simulink model "ASM_Traffic_new"  (R2024a)
settings: Solver=ode1  StartTime=SIM.tstart.v  StopTime=SIM.tend.v  FixedStep=SIM.StepSize.v  RelTol=1e-3
PostLoadFcn:
  | if any(exist('dsrtsu_mdlpostloadfcn', 'file') ~= 0), dsrtsu_mdlpostloadfcn('Execute', bdroot); end
  | try, asm_mdl_postloadfcn(bdroot, 'UpdateModel', 3600); catch, disp(lasterr); end,
InitFcn:
  | , if any(exist('rtifpga_mdlclblib', 'file') ~= 0), rtifpga_mdlclblib('Init', bdroot); end,
  | , if any(exist('dsmpb_private', 'file') ~= 0), dsmpb_private('dsmpb_mdlclblib', 'Init', bdroot); end,
undefined symbols (not defined in the file): _to_, a0b2, ASM_BrakeHydraulics_DemoSystems, ASM_VehicleDynamics_DemoSystems, b98103fe8ad365046cd0, BrakeCircuit, CPT, Crankshaft, DiscIntNeverNeededParam, dsmsi, FinalDriveAssembly, MDL, ModeSignals, Pos_BrakePedal_Maneuver, rad, RefSignals, s_to_rpm, SIM, SoftECU, Suspension, Tire, Transmission
libraries: ASM_Traffic_lib x135, simulink x100, ASM_Utils_lib x77, ASM_VehicleDynamics_lib x70, ASM_Environment_lib x22, dsmpblib x20, dsmsilib x15, MDLD_Utils_lib x10, ASM_BrakeHydraulics_lib x3
(part 42 of 63)

== system ASM_Traffic_new/VehicleDynamics/Plant/UserInterface/DISP_Plant/Aerodynamics ==
  Aerodynamics : Inport
  Aerodynamics1 : Scope  NumInputPorts=2
  Bus Selector5 : BusSelector  OutputSignals=Forces.F_x_Aero_CoorSys_V[N],Forces.F_y_Aero_CoorSys_V[N],Forces.F_z_Aero_CoorSys_V[N],Torques.Trq_x_Aero_CoorSys_V[Nm],Torques.Trq_y_Aero_CoorSys_V[Nm],Torques.Trq_z_Aero_CoorSys_V[Nm]
  F_x_Aero_CoorSys_V[N] : Subsystem
      mask Display: disp('')
  F_y_Aero_CoorSys_V[N] : Subsystem
      mask Display: disp('')
  F_z_Aero_CoorSys_V[N] : Subsystem
      mask Display: disp('')
  Mux : Mux  Inputs=3
  Mux1 : Mux  Inputs=3
  Trq_x_Aero_CoorSys_V[Nm] : Subsystem
      mask Display: disp('')
  Trq_y_Aero_CoorSys_V[Nm] : Subsystem
      mask Display: disp('')
  Trq_z_Aero_CoorSys_V[Nm] : Subsystem
      mask Display: disp('')
  wires:
  Trq_z_Aero_CoorSys_V[Nm]/1(Out1) -> Mux1/3  "Trq_z_Aero_CoorSys_V[Nm]"
  Bus Selector5/6 -> Trq_z_Aero_CoorSys_V[Nm]/1(In1)  "<Trq_z_Aero_CoorSys_V[Nm]>"
  Trq_y_Aero_CoorSys_V[Nm]/1(Out1) -> Mux1/2  "Trq_y_Aero_CoorSys_V[Nm]"
  Bus Selector5/5 -> Trq_y_Aero_CoorSys_V[Nm]/1(In1)  "<Trq_y_Aero_CoorSys_V[Nm]>"
  Trq_x_Aero_CoorSys_V[Nm]/1(Out1) -> Mux1/1  "Trq_x_Aero_CoorSys_V[Nm]"
  Bus Selector5/4 -> Trq_x_Aero_CoorSys_V[Nm]/1(In1)  "<Trq_x_Aero_CoorSys_V[Nm]>"
  F_z_Aero_CoorSys_V[N]/1(Out1) -> Mux/3  "F_z_Aero_CoorSys_V[N]"
  Bus Selector5/3 -> F_z_Aero_CoorSys_V[N]/1(In1)  "<F_z_Aero_CoorSys_V[N]>"
  F_y_Aero_CoorSys_V[N]/1(Out1) -> Mux/2  "F_y_Aero_CoorSys_V[N]"
  Bus Selector5/2 -> F_y_Aero_CoorSys_V[N]/1(In1)  "<F_y_Aero_CoorSys_V[N]>"
  F_x_Aero_CoorSys_V[N]/1(Out1) -> Mux/1  "F_x_Aero_CoorSys_V[N]"
  Bus Selector5/1 -> F_x_Aero_CoorSys_V[N]/1(In1)  "<F_x_Aero_CoorSys_V[N]>"
  Mux1/1 -> Aerodynamics1/2  "Trq_Aero[Nm]"
  Mux/1 -> Aerodynamics1/1  "F_Aero[N]"
  Aerodynamics/1 -> Bus Selector5/1

== system ASM_Traffic_new/VehicleDynamics/Plant/UserInterface/DISP_Plant/Brake ==
  Brake : Inport
  BrakeHydraulicsModel : Display
      settings: AttributesFormatString=1 - Complex\n2 - Basic
  BrakeHydraulicsModel[] : Subsystem
      mask Display: disp('')
  BrakePressure : Scope  NumInputPorts=6
  BrakeTorques : Scope  NumInputPorts=4
  Bus Selector2 : BusSelector  OutputSignals=BrakeHydraulics.BrakeHydraulicsModel[],BrakeDisc.Torque.Trq_FL_Brake[Nm],BrakeDisc.Torque.Trq_FR_Brake[Nm],BrakeDisc.Torque.Trq_RL_Brake[Nm],BrakeDisc.Torque.Trq_RR_Brake[Nm],MasterBrakeCylinder.ActiveBrakeCylinder.p[bar],MasterBrakeCylinder.ActiveBrakeCylinder.p_max[bar],BrakeDisc.Pressure.p_FL_Brake[bar],BrakeDisc.Pressure.p_FR_Brake[bar],BrakeDisc.Pressure.p_RL_Brake[bar],BrakeDisc.Pressure.p_RR_Brake[bar]
  Trq_FL_Brake[Nm] : Subsystem
      mask Display: disp('')
  Trq_FR_Brake[Nm] : Subsystem
      mask Display: disp('')
  Trq_RL_Brake[Nm] : Subsystem
      mask Display: disp('')
  Trq_RR_Brake[Nm] : Subsystem
      mask Display: disp('')
  p[bar] : Subsystem
      mask Display: disp('')
  p_FL_Brake[bar] : Subsystem
      mask Display: disp('')
  p_FR_Brake[bar] : Subsystem
      mask Display: disp('')
  p_RL_Brake[bar] : Subsystem
      mask Display: disp('')
  p_RR_Brake[bar] : Subsystem
      mask Display: disp('')
  p_max[bar] : Subsystem
      mask Display: disp('')
  wires:
  p_RR_Brake[bar]/1(Out1) -> BrakePressure/6  "p_RR_Brake[bar]"
  Bus Selector2/11 -> p_RR_Brake[bar]/1(In1)  "<p_RR_Brake[bar]>"
  p_RL_Brake[bar]/1(Out1) -> BrakePressure/5  "p_RL_Brake[bar]"
  Bus Selector2/10 -> p_RL_Brake[bar]/1(In1)  "<p_RL_Brake[bar]>"
  p_FR_Brake[bar]/1(Out1) -> BrakePressure/4  "p_FR_Brake[bar]"
  Bus Selector2/9 -> p_FR_Brake[bar]/1(In1)  "<p_FR_Brake[bar]>"
  p_FL_Brake[bar]/1(Out1) -> BrakePressure/3  "p_FL_Brake[bar]"
  Bus Selector2/8 -> p_FL_Brake[bar]/1(In1)  "<p_FL_Brake[bar]>"
  p_max[bar]/1(Out1) -> BrakePressure/2  "p_max[bar]"
  Bus Selector2/7 -> p_max[bar]/1(In1)  "<p_max[bar]>"
  p[bar]/1(Out1) -> BrakePressure/1  "p[bar]"
  Bus Selector2/6 -> p[bar]/1(In1)  "<p[bar]>"
  Trq_RR_Brake[Nm]/1(Out1) -> BrakeTorques/4  "Trq_RR_Brake[Nm]"
  Bus Selector2/5 -> Trq_RR_Brake[Nm]/1(In1)  "<Trq_RR_Brake[Nm]>"
  Trq_RL_Brake[Nm]/1(Out1) -> BrakeTorques/3  "Trq_RL_Brake[Nm]"
  Bus Selector2/4 -> Trq_RL_Brake[Nm]/1(In1)  "<Trq_RL_Brake[Nm]>"
  Trq_FR_Brake[Nm]/1(Out1) -> BrakeTorques/2  "Trq_FR_Brake[Nm]"
  Bus Selector2/3 -> Trq_FR_Brake[Nm]/1(In1)  "<Trq_FR_Brake[Nm]>"
  Trq_FL_Brake[Nm]/1(Out1) -> BrakeTorques/1  "Trq_FL_Brake[Nm]"
  Bus Selector2/2 -> Trq_FL_Brake[Nm]/1(In1)  "<Trq_FL_Brake[Nm]>"
  Brake/1 -> Bus Selector2/1
  BrakeHydraulicsModel[]/1(Out1) -> BrakeHydraulicsModel/1  "BrakeHydraulicsModel[]"
  Bus Selector2/1 -> BrakeHydraulicsModel[]/1(In1)  "<BrakeHydraulicsModel[]>"

== system ASM_Traffic_new/VehicleDynamics/Plant/UserInterface/DISP_Plant/Overview ==
  Velocities : Inport
  Accelerations : Inport  Port=2
  Bus Selector1 : BusSelector  OutputSignals=VehicleCoG.Linear.a_Vehicle_CoG[x;y;z][m|s2].a_x_Vehicle_CoG[m|s2],VehicleCoG.Linear.a_Vehicle_CoG[x;y;z][m|s2].a_y_Vehicle_CoG[m|s2],VehicleCoG.Linear.a_Vehicle_CoG[x;y;z][m|s2].a_z_Vehicle_CoG[m|s2]
  Bus Selector2 : BusSelector  OutputSignals=Vehicle.Linear.v_Vehicle_CoG[x;y;z][km|h].v_x_Vehicle_CoG[km|h],Vehicle.Linear.v_Vehicle_CoG[x;y;z][km|h].v_y_Vehicle_CoG[km|h],Vehicle.Linear.v_Vehicle_CoG[x;y;z][km|h].v_z_Vehicle_CoG[km|h],Vehicle.Linear.v_Total_Vehicle[km|h]
  Mux : Mux
  Mux1 : Mux  Inputs=3
  Overview : Scope  NumInputPorts=2
  a_x_Vehicle_CoG[m|s2] : Subsystem
      mask Display: disp('')
  a_y_Vehicle_CoG[m|s2] : Subsystem
      mask Display: disp('')
  a_z_Vehicle_CoG[m|s2] : Subsystem
      mask Display: disp('')
  v_Total_Vehicle[km|h] : Subsystem
      mask Display: disp('')
  v_x_Vehicle_CoG[km|h] : Subsystem
      mask Display: disp('')
  v_y_Vehicle_CoG[km|h] : Subsystem
      mask Display: disp('')
  v_z_Vehicle_CoG[km|h] : Subsystem
      mask Display: disp('')
  wires:
  Velocities/1 -> Bus Selector2/1
  Accelerations/1 -> Bus Selector1/1
  Mux/1 -> Overview/1  "Velocities"
  Mux1/1 -> Overview/2  "Accelerations"
  v_x_Vehicle_CoG[km|h]/1(Out1) -> Mux/1  "v_x_Vehicle_CoG[km|h]"
  v_y_Vehicle_CoG[km|h]/1(Out1) -> Mux/2  "v_y_Vehicle_CoG[km|h]"
  v_z_Vehicle_CoG[km|h]/1(Out1) -> Mux/3  "v_z_Vehicle_CoG[km|h]"
  v_Total_Vehicle[km|h]/1(Out1) -> Mux/4  "v_Total_Vehicle[km|h]"
  a_x_Vehicle_CoG[m|s2]/1(Out1) -> Mux1/1  "a_x_Vehicle_CoG[m|s2]"
  a_y_Vehicle_CoG[m|s2]/1(Out1) -> Mux1/2  "a_y_Vehicle_CoG[m|s2]"
  a_z_Vehicle_CoG[m|s2]/1(Out1) -> Mux1/3  "a_z_Vehicle_CoG[m|s2]"
  Bus Selector2/1 -> v_x_Vehicle_CoG[km|h]/1(In1)  "<v_x_Vehicle_CoG[km|h]>"
  Bus Selector2/2 -> v_y_Vehicle_CoG[km|h]/1(In1)  "<v_y_Vehicle_CoG[km|h]>"
  Bus Selector2/3 -> v_z_Vehicle_CoG[km|h]/1(In1)  "<v_z_Vehicle_CoG[km|h]>"
  Bus Selector2/4 -> v_Total_Vehicle[km|h]/1(In1)  "<v_Total_Vehicle[km|h]>"
  Bus Selector1/1 -> a_x_Vehicle_CoG[m|s2]/1(In1)  "<a_x_Vehicle_CoG[m|s2]>"
  Bus Selector1/2 -> a_y_Vehicle_CoG[m|s2]/1(In1)  "<a_y_Vehicle_CoG[m|s2]>"
  Bus Selector1/3 -> a_z_Vehicle_CoG[m|s2]/1(In1)  "<a_z_Vehicle_CoG[m|s2]>"

== system ASM_Traffic_new/VehicleDynamics/Plant/UserInterface/DISP_Plant/Positions ==
  Positions : Inport
  Angle_Pitch_Vehicle_CoorSys_E[deg] : Subsystem
      mask Display: disp('')
  Angle_Roll_Vehicle_CoorSys_E[deg] : Subsystem
      mask Display: disp('')
  Angle_Yaw_Vehicle_CoorSys_E[deg] : Subsystem
      mask Display: disp('')
  AngularPosition : Scope  NumInputPorts=3
  Bus Selector2 : BusSelector  OutputSignals=Vehicle.Linear.Pos_Vehicle_CoorSys_E[m],Vehicle.Linear.s_Vehicle[m],Vehicle.Angular.Angle_V[Alpha;Beta;Gamma][deg]
  Demux : Demux  Outputs=3
  Demux1 : Demux  Outputs=3
  Pos_x_Vehicle_CoorSys_E[m] : Subsystem
      mask Display: disp('')
  Pos_y_Vehicle_CoorSys_E[m] : Subsystem
      mask Display: disp('')
  Pos_z_Vehicle_CoorSys_E[m] : Subsystem
      mask Display: disp('')
  TransPosition : Scope  NumInputPorts=4
  s_Vehicle[m] : Subsystem
      mask Display: disp('')
  wires:
  Positions/1 -> Bus Selector2/1
  Angle_Roll_Vehicle_CoorSys_E[deg]/1(Out1) -> AngularPosition/1  "Angle_Roll_Vehicle_CoorSys_E[deg]"
  Angle_Pitch_Vehicle_CoorSys_E[deg]/1(Out1) -> AngularPosition/2  "Angle_Pitch_Vehicle_CoorSys_E[deg]"
  Angle_Yaw_Vehicle_CoorSys_E[deg]/1(Out1) -> AngularPosition/3  "Angle_Yaw_Vehicle_CoorSys_E[deg]"
  Pos_x_Vehicle_CoorSys_E[m]/1(Out1) -> TransPosition/1  "Pos_x_Vehicle_CoorSys_E[m]"
  Pos_y_Vehicle_CoorSys_E[m]/1(Out1) -> TransPosition/2  "Pos_y_Vehicle_CoorSys_E[m]"
  Pos_z_Vehicle_CoorSys_E[m]/1(Out1) -> TransPosition/3  "Pos_z_Vehicle_CoorSys_E[m]"
  s_Vehicle[m]/1(Out1) -> TransPosition/4  "s_Vehicle[m]"
  Bus Selector2/1 -> Demux/1  "<Pos_Vehicle_CoorSys_E[m]>"
  Bus Selector2/2 -> s_Vehicle[m]/1(In1)  "<s_Vehicle[m]>"
  Demux/1 -> Pos_x_Vehicle_CoorSys_E[m]/1(In1)
  Demux/2 -> Pos_y_Vehicle_CoorSys_E[m]/1(In1)
  Demux/3 -> Pos_z_Vehicle_CoorSys_E[m]/1(In1)
  Demux1/2 -> Angle_Pitch_Vehicle_CoorSys_E[deg]/1(In1)
  Demux1/1 -> Angle_Roll_Vehicle_CoorSys_E[deg]/1(In1)
  Demux1/3 -> Angle_Yaw_Vehicle_CoorSys_E[deg]/1(In1)
  Bus Selector2/3 -> Demux1/1  "<Angle_V[Alpha;Beta;Gamma][deg]>"

== system ASM_Traffic_new/VehicleDynamics/Plant/UserInterface/DISP_Plant/Sensor1 ==
  Sensor1 : Inport
  AngularAccelerations : Scope
  AngularVelocity : Scope
  AngularVelocity_CoorSys_VH : Scope
  Bus Selector2 : BusSelector  OutputSignals=a_Angular_Sensor1_CoorSys_V[x;y;z][rad|s2],a_Total_Sensor1_CoorSys_V[x;y;z][m|s2],a_Sensor1_CoorSys_V[x;y;z][m|s2],v_Sensor1_CoorSys_V[x;y;z][m|s],w_Sensor1_CoorSys_V[x;y;z][rad|s],a_Angular_Sensor1_CoorSys_VH[x;y;z][rad|s2],a_Total_Sensor1_CoorSys_VH[x;y;z][m|s2],a_Sensor1_CoorSys_VH[x;y;z][m|s2],v_Sensor1_CoorSys_VH[x;y;z][m|s],w_Sensor1_CoorSys_VH[x;y;z][rad|s]
  TransAccelerations_CoorSys_VH : Scope
  TransAccelerations_withGravity : Scope
  TransAccelerations_withGravity_CoorSys_VH : Scope
  TransAccelerations_withoutGravity : Scope
  TransAccelerations_withoutGravity_CoorSys_VH : Scope
  TransVelocity : Scope
  TransVelocity_CoorSys_VH : Scope
  a_Angular_Sensor1_CoorSys_VH[x;y;z][rad|s2] : Subsystem
      mask Display: disp('')
  a_Angular_Sensor1_CoorSys_V[x;y;z][rad|s2] : Subsystem
      mask Display: disp('')
  a_Sensor1_CoorSys_VH[x;y;z][m|s2] : Subsystem
      mask Display: disp('')
  a_Sensor1_CoorSys_V[x;y;z][m|s2] : Subsystem
      mask Display: disp('')
  a_Total_Sensor1_CoorSys_VH[x;y;z][m|s2] : Subsystem
      mask Display: disp('')
  a_Total_Sensor1_CoorSys_V[x;y;z][m|s2] : Subsystem
      mask Display: disp('')
  v_Sensor1_CoorSys_VH[x;y;z][m|s] : Subsystem
      mask Display: disp('')
  v_Sensor1_CoorSys_V[x;y;z][m|s] : Subsystem
      mask Display: disp('')
  w_Sensor1_CoorSys_VH[x;y;z][rad|s] : Subsystem
      mask Display: disp('')
  w_Sensor1_CoorSys_V[x;y;z][rad|s] : Subsystem
      mask Display: disp('')
  wires:
  Bus Selector2/9 -> v_Sensor1_CoorSys_VH[x;y;z][m|s]/1(In1)  "<v_Sensor1_CoorSys_VH[x;y;z][m|s]>"
  v_Sensor1_CoorSys_VH[x;y;z][m|s]/1(Out1) -> TransVelocity_CoorSys_VH/1  "v_Sensor1_CoorSys_VH[x;y;z][m|s]"
  w_Sensor1_CoorSys_VH[x;y;z][rad|s]/1(Out1) -> AngularVelocity_CoorSys_VH/1  "w_Sensor1_CoorSys_VH[x;y;z][rad|s]"
  Bus Selector2/10 -> w_Sensor1_CoorSys_VH[x;y;z][rad|s]/1(In1)  "<w_Sensor1_CoorSys_VH[x;y;z][rad|s]>"
  Bus Selector2/7 -> a_Total_Sensor1_CoorSys_VH[x;y;z][m|s2]/1(In1)  "<a_Total_Sensor1_CoorSys_VH[x;y;z][m|s2]>"
  a_Total_Sensor1_CoorSys_VH[x;y;z][m|s2]/1(Out1) -> TransAccelerations_withGravity_CoorSys_VH/1  "a_Total_Sensor1_CoorSys_VH[x;y;z][m|s2]"
  a_Sensor1_CoorSys_VH[x;y;z][m|s2]/1(Out1) -> TransAccelerations_withoutGravity_CoorSys_VH/1  "a_Sensor1_CoorSys_VH[x;y;z][m|s2]"
  Bus Selector2/8 -> a_Sensor1_CoorSys_VH[x;y;z][m|s2]/1(In1)  "<a_Sensor1_CoorSys_VH[x;y;z][m|s2]>"
  Bus Selector2/5 -> w_Sensor1_CoorSys_V[x;y;z][rad|s]/1(In1)  "<w_Sensor1_CoorSys_V[x;y;z][rad|s]>"
  w_Sensor1_CoorSys_V[x;y;z][rad|s]/1(Out1) -> AngularVelocity/1  "w_Sensor1_CoorSys_V[x;y;z][rad|s]"
  a_Angular_Sensor1_CoorSys_VH[x;y;z][rad|s2]/1(Out1) -> TransAccelerations_CoorSys_VH/1  "a_Angular_Sensor1_CoorSys_VH[x;y;z][rad|s2]"
  Bus Selector2/6 -> a_Angular_Sensor1_CoorSys_VH[x;y;z][rad|s2]/1(In1)  "<a_Angular_Sensor1_CoorSys_VH[x;y;z][rad|s2]>"
  Bus Selector2/3 -> a_Sensor1_CoorSys_V[x;y;z][m|s2]/1(In1)  "<a_Sensor1_CoorSys_V[x;y;z][m|s2]>"
  a_Sensor1_CoorSys_V[x;y;z][m|s2]/1(Out1) -> TransAccelerations_withoutGravity/1  "a_Sensor1_CoorSys_V[x;y;z][m|s2]"
  v_Sensor1_CoorSys_V[x;y;z][m|s]/1(Out1) -> TransVelocity/1  "v_Sensor1_CoorSys_V[x;y;z][m|s]"
  Bus Selector2/4 -> v_Sensor1_CoorSys_V[x;y;z][m|s]/1(In1)  "<v_Sensor1_CoorSys_V[x;y;z][m|s]>"
  a_Total_Sensor1_CoorSys_V[x;y;z][m|s2]/1(Out1) -> TransAccelerations_withGravity/1  "a_Total_Sensor1_CoorSys_V[x;y;z][m|s2]"
  Bus Selector2/2 -> a_Total_Sensor1_CoorSys_V[x;y;z][m|s2]/1(In1)  "<a_Total_Sensor1_CoorSys_V[x;y;z][m|s2]>"
  a_Angular_Sensor1_CoorSys_V[x;y;z][rad|s2]/1(Out1) -> AngularAccelerations/1  "a_Angular_Sensor1_CoorSys_V[x;y;z][rad|s2]"
  Bus Selector2/1 -> a_Angular_Sensor1_CoorSys_V[x;y;z][rad|s2]/1(In1)  "<a_Angular_Sensor1_CoorSys_V[x;y;z][rad|s2]>"
  Sensor1/1 -> Bus Selector2/1

== system ASM_Traffic_new/VehicleDynamics/Plant/UserInterface/DISP_Plant/Steering ==
  Steering : Inport
  Angle_SteeringGear[deg] : Subsystem
      mask Display: disp('')
  Angle_SteeringWheel[deg] : Subsystem
      mask Display: disp('')
  Bus Selector2 : BusSelector  OutputSignals=Displ_Steering[m],i_Steering_Mean[],ForcesAndTorques.TrqSpring_SteeringColumn[Nm],ForcesAndTorques.Trq_PowerSteering[Nm],Angle_SteeringWheel[deg],Angle_SteeringGear[deg]
  Displ_Steering[m] : Subsystem
      mask Display: disp('')
  SteeringSignals : Scope  NumInputPorts=6
  Trq_PowerSteering[Nm] : Subsystem
      mask Display: disp('')
  Trq_Steering[Nm] : Subsystem
      mask Display: disp('')
  i_Steering_Mean[] : Subsystem
      mask Display: disp('')
  wires:
  Steering/1 -> Bus Selector2/1
  Displ_Steering[m]/1(Out1) -> SteeringSignals/1  "Displ_Steering[m]"
  i_Steering_Mean[]/1(Out1) -> SteeringSignals/2  "i_Steering_Mean[]"
  Trq_Steering[Nm]/1(Out1) -> SteeringSignals/3  "Trq_Steering[Nm]"
  Trq_PowerSteering[Nm]/1(Out1) -> SteeringSignals/4  "Trq_PowerSteering[Nm]"
  Bus Selector2/1 -> Displ_Steering[m]/1(In1)  "<Displ_Steering[m]>"
  Bus Selector2/2 -> i_Steering_Mean[]/1(In1)  "<i_Steering_Mean[]>"
  Bus Selector2/3 -> Trq_Steering[Nm]/1(In1)  "<TrqSpring_SteeringColumn[Nm]>"
  Bus Selector2/4 -> Trq_PowerSteering[Nm]/1(In1)  "<Trq_PowerSteering[Nm]>"
  Bus Selector2/5 -> Angle_SteeringWheel[deg]/1(In1)  "<Angle_SteeringWheel[deg]>"
  Bus Selector2/6 -> Angle_SteeringGear[deg]/1(In1)  "<Angle_SteeringGear[deg]>"
  Angle_SteeringWheel[deg]/1(Out1) -> SteeringSignals/5  "Angle_SteeringWheel[deg]"
  Angle_SteeringGear[deg]/1(Out1) -> SteeringSignals/6  "Angle_SteeringGear[deg]"

== system ASM_Traffic_new/VehicleDynamics/Plant/UserInterface/DISP_Plant/Suspension ==
  Suspension : Inport
  Angle_Alpha_FL_Wheel[deg] : Subsystem
      mask Display: disp('')
  Angle_Alpha_FR_Wheel[deg] : Subsystem
      mask Display: disp('')
  Angle_Alpha_RL_Wheel[deg] : Subsystem
      mask Display: disp('')
  Angle_Alpha_RR_Wheel[deg] : Subsystem
      mask Display: disp('')
  Angle_Beta_FL_Wheel[deg] : Subsystem
      mask Display: disp('')
  Angle_Beta_FR_Wheel[deg] : Subsystem
      mask Display: disp('')
  Angle_Beta_RL_Wheel[deg] : Subsystem
      mask Display: disp('')
  Angle_Beta_RR_Wheel[deg] : Subsystem
      mask Display: disp('')
  Angle_FL_Wheel[Alpha;Beta;Gamma][deg] : Subsystem
      mask Display: disp('')
  Angle_FRWheel[Alpha;Beta;Gamma][deg] : Subsystem
      mask Display: disp('')
  Angle_Gamma_FL_Wheel[deg] : Subsystem
      mask Display: disp('')
  Angle_Gamma_FR_Wheel[deg] : Subsystem
      mask Display: disp('')
  Angle_Gamma_RL_Wheel[deg] : Subsystem
      mask Display: disp('')
  Angle_Gamma_RR_Wheel[deg] : Subsystem
      mask Display: disp('')
  Angle_RL_Wheel[Alpha;Beta;Gamma][deg] : Subsystem
      mask Display: disp('')
  Angle_RR_Wheel[Alpha;Beta;Gamma][deg] : Subsystem
      mask Display: disp('')
  Bus Selector : BusSelector  OutputSignals=Kinematics_Left.Position_Left.Pos_Left_Wheel[x;y;z][m],Kinematics_Left.Orientation_Left.Angle_Left_Wheel[Alpha;Beta;Gamma][deg],Kinematics_Left.Orientation_Left.Angle_Left_Wheel[Alpha;Beta;Gamma][deg].Angle_Alpha_Left_Wheel[deg],Kinematics_Left.Orientation_Left.Angle_Left_Wheel[Alpha;Beta;Gamma][deg].Angle_Beta_Left_Wheel[deg],Kinematics_Left.Orientation_Left.Angle_Left_Wheel[Alpha;Beta;Gamma][deg].Angle_Gamma_Left_Wheel[deg],Kinematics_Left.Spring_Left.Displ_Spring_Left[m],Kinematics_Left.Damper_Left.Displ_Damper_Left[m],Kinematics_Left.Damper_Left.Displ_Damper_Left_dt[m|s],Kinematics_Right.Position_Right.Pos_Right_Wheel[x;y;z][m],Kinematics_Right.Orientation_Right.Angle_Right_Wheel[Alpha;Beta;Gamma][deg],Kinematics_Right.Orientation_Right.Angle_Right_Wheel[Alpha;Beta;Gamma][deg].Angle_Alpha_Right_Wheel[deg],Kinematics_Right.Orientation_Right.Angle_Right_Wheel[Alpha;Beta;Gamma][deg].Angle_Beta_Right_Wheel[deg],Kinematics_Right.Orientation_Right.Angle_Right_Wheel[Alpha;Beta;Gamma][deg].Angle_Gamma_Right_Wheel[deg],Kinematics_Right.Spring_Right.Displ_Spring_Right[m],Kinematics_Right.Damper_Right.Displ_Damper_Right[m],Kinematics_Right.Damper_Right.Displ_Damper_Right_dt[m|s],Stabilizer.Displ_Stabilizer[m]
  Bus Selector1 : BusSelector  OutputSignals=SuspensionFront.SuspensionKinematicsFront,SuspensionFront.SuspensionForcesFront,SuspensionRear.SuspensionKinematicsRear,SuspensionRear.SuspensionForcesRear
  Bus Selector2 : BusSelector  OutputSignals=Kinematics_Left.Position_Left.Pos_Left_Wheel[x;y;z][m],Kinematics_Left.Orientation_Left.Angle_Left_Wheel[Alpha;Beta;Gamma][deg],Kinematics_Left.Orientation_Left.Angle_Left_Wheel[Alpha;Beta;Gamma][deg].Angle_Alpha_Left_Wheel[deg],Kinematics_Left.Orientation_Left.Angle_Left_Wheel[Alpha;Beta;Gamma][deg].Angle_Beta_Left_Wheel[deg],Kinematics_Left.Orientation_Left.Angle_Left_Wheel[Alpha;Beta;Gamma][deg].Angle_Gamma_Left_Wheel[deg],Kinematics_Left.Spring_Left.Displ_Spring_Left[m],Kinematics_Left.Damper_Left.Displ_Damper_Left[m],Kinematics_Left.Damper_Left.Displ_Damper_Left_dt[m|s],Kinematics_Right.Position_Right.Pos_Right_Wheel[x;y;z][m],Kinematics_Right.Orientation_Right.Angle_Right_Wheel[Alpha;Beta;Gamma][deg],Kinematics_Right.Orientation_Right.Angle_Right_Wheel[Alpha;Beta;Gamma][deg].Angle_Alpha_Right_Wheel[deg],Kinematics_Right.Orientation_Right.Angle_Right_Wheel[Alpha;Beta;Gamma][deg].Angle_Beta_Right_Wheel[deg],Kinematics_Right.Orientation_Right.Angle_Right_Wheel[Alpha;Beta;Gamma][deg].Angle_Gamma_Right_Wheel[deg],Kinematics_Right.Spring_Right.Displ_Spring_Right[m],Kinematics_Right.Damper_Right.Displ_Damper_Right[m],Kinematics_Right.Damper_Right.Displ_Damper_Right_dt[m|s],Stabilizer.Displ_Stabilizer[m]
  Bus Selector3 : BusSelector  OutputSignals=F_FL_Spring[N],F_FL_Damper[N],F_FR_Spring[N],F_FR_Damper[N],F_Stabilizer[N]
  Bus Selector4 : BusSelector  OutputSignals=F_RL_Spring[N],F_RL_Damper[N],F_RR_Spring[N],F_RR_Damper[N],F_Stabilizer[N]
  Displ_Damper_FL[m] : Subsystem
      mask Display: disp('')
  Displ_Damper_FL_dt[m|s] : Subsystem
      mask Display: disp('')
  Displ_Damper_FR[m] : Subsystem
      mask Display: disp('')
  Displ_Damper_FR_dt[m|s] : Subsystem
      mask Display: disp('')
  Displ_Damper_RL[m] : Subsystem
      mask Display: disp('')
  Displ_Damper_RL_dt[m|s] : Subsystem
      mask Display: disp('')
  Displ_Damper_RR[m] : Subsystem
      mask Display: disp('')
  Displ_Damper_RR_dt[m|s] : Subsystem
      mask Display: disp('')
  Displ_Spring_FL[m] : Subsystem
      mask Display: disp('')
  Displ_Spring_FRm] : Subsystem
      mask Display: disp('')
  Displ_Spring_RL[m] : Subsystem
      mask Display: disp('')
  Displ_Spring_RR[m] : Subsystem
      mask Display: disp('')
  Displ_Stabilizer_Front[m] : Subsystem
      mask Display: disp('')
  Displ_Stabilizer_Rear[m] : Subsystem
      mask Display: disp('')
  F_FL_Damper[N] : Subsystem
      mask Display: disp('')
  F_FL_Spring[N] : Subsystem
      mask Display: disp('')
  F_FR_Damper[N] : Subsystem
      mask Display: disp('')
  F_FR_Spring[N] : Subsystem
      mask Display: disp('')
  F_RL_Damper[N] : Subsystem
      mask Display: disp('')
  F_RL_Spring[N] : Subsystem
      mask Display: disp('')
  F_RR_Damper[N] : Subsystem
      mask Display: disp('')
  F_RR_Spring[N] : Subsystem
      mask Display: disp('')
  F_Stabilizer_Front[N] : Subsystem
      mask Display: disp('')
  F_Stabilizer_Rear[N] : Subsystem
      mask Display: disp('')
  Force_Front : Scope  NumInputPorts=5
  Force_Rear : Scope  NumInputPorts=5
  Kin_FL : Scope  NumInputPorts=5
  Kin_FR : Scope  NumInputPorts=5
  Kin_RL : Scope  NumInputPorts=5
  Kin_RR : Scope  NumInputPorts=5
  Kin_Stabi_Front : Scope
  Kin_Stabi_Rear : Scope
  Mux{,1..3} (4 alike) : Mux  Inputs=3
  Pos_FL_Wheel[x;y;z][m] : Subsystem
      mask Display: disp('')
  Pos_FR_Wheel[x;y;z][m] : Subsystem
      mask Display: disp('')
  Pos_RL_Wheel[x;y;z][m] : Subsystem
      mask Display: disp('')
  Pos_RR_Wheel[x;y;z][m] : Subsystem
      mask Display: disp('')
  Terminator{,1..3} (4 alike) : Terminator
  wires:
  Bus Selector/13 -> Angle_Gamma_FR_Wheel[deg]/1(In1)  "<Angle_Gamma_Right_Wheel[deg]>"
  Bus Selector/12 -> Angle_Beta_FR_Wheel[deg]/1(In1)  "<Angle_Beta_Right_Wheel[deg]>"
  Bus Selector/11 -> Angle_Alpha_FR_Wheel[deg]/1(In1)  "<Angle_Alpha_Right_Wheel[deg]>"
  Angle_FRWheel[Alpha;Beta;Gamma][deg]/1(Out1) -> Terminator3/1
  Mux3/1 -> Kin_FR/2  "Angle_FR_Wheel[Alpha;Beta;Gamma][deg]"
  Angle_Gamma_FR_Wheel[deg]/1(Out1) -> Mux3/3
  Angle_Beta_FR_Wheel[deg]/1(Out1) -> Mux3/2
  Angle_Alpha_FR_Wheel[deg]/1(Out1) -> Mux3/1
  Bus Selector/14 -> Displ_Spring_FRm]/1(In1)  "<Displ_Spring_Right[m]>"
  Bus Selector/15 -> Displ_Damper_FR[m]/1(In1)  "<Displ_Damper_Right[m]>"
  Bus Selector/16 -> Displ_Damper_FR_dt[m|s]/1(In1)  "<Displ_Damper_Right_dt[m|s]>"
  Bus Selector/17 -> Displ_Stabilizer_Front[m]/1(In1)  "<Displ_Stabilizer[m]>"
  Bus Selector/10 -> Angle_FRWheel[Alpha;Beta;Gamma][deg]/1(In1)  "<Angle_Right_Wheel[Alpha;Beta;Gamma][deg]>"
  Bus Selector/9 -> Pos_FR_Wheel[x;y;z][m]/1(In1)  "<Pos_Right_Wheel[x;y;z][m]>"
  Bus Selector/8 -> Displ_Damper_FL_dt[m|s]/1(In1)  "<Displ_Damper_Left_dt[m|s]>"
  Bus Selector/7 -> Displ_Damper_FL[m]/1(In1)  "<Displ_Damper_Left[m]>"
  Bus Selector/6 -> Displ_Spring_FL[m]/1(In1)  "<Displ_Spring_Left[m]>"
  Bus Selector/5 -> Angle_Gamma_FL_Wheel[deg]/1(In1)  "<Angle_Gamma_Left_Wheel[deg]>"
  Bus Selector/4 -> Angle_Beta_FL_Wheel[deg]/1(In1)  "<Angle_Beta_Left_Wheel[deg]>"
  Bus Selector/3 -> Angle_Alpha_FL_Wheel[deg]/1(In1)  "<Angle_Alpha_Left_Wheel[deg]>"
  Mux2/1 -> Kin_FL/2  "Angle_FL_Wheel[Alpha;Beta;Gamma][deg]"
  Angle_FL_Wheel[Alpha;Beta;Gamma][deg]/1(Out1) -> Terminator2/1
  Angle_Gamma_FL_Wheel[deg]/1(Out1) -> Mux2/3
  Angle_Beta_FL_Wheel[deg]/1(Out1) -> Mux2/2
  Angle_Alpha_FL_Wheel[deg]/1(Out1) -> Mux2/1
  Bus Selector/2 -> Angle_FL_Wheel[Alpha;Beta;Gamma][deg]/1(In1)  "<Angle_Left_Wheel[Alpha;Beta;Gamma][deg]>"
  Angle_RL_Wheel[Alpha;Beta;Gamma][deg]/1(Out1) -> Terminator1/1
  Bus Selector2/5 -> Angle_Gamma_RL_Wheel[deg]/1(In1)  "<Angle_Gamma_Left_Wheel[deg]>"
  Bus Selector2/4 -> Angle_Beta_RL_Wheel[deg]/1(In1)  "<Angle_Beta_Left_Wheel[deg]>"
  Bus Selector2/3 -> Angle_Alpha_RL_Wheel[deg]/1(In1)  "<Angle_Alpha_Left_Wheel[deg]>"
  Mux1/1 -> Kin_RL/2  "Angle_RL_Wheel[Alpha;Beta;Gamma][deg]"
  Angle_Gamma_RL_Wheel[deg]/1(Out1) -> Mux1/3
  Angle_Beta_RL_Wheel[deg]/1(Out1) -> Mux1/2
  Angle_Alpha_RL_Wheel[deg]/1(Out1) -> Mux1/1
  Angle_RR_Wheel[Alpha;Beta;Gamma][deg]/1(Out1) -> Terminator/1
  Mux/1 -> Kin_RR/2  "Angle_RR_Wheel[Alpha;Beta;Gamma][deg]"
  Angle_Gamma_RR_Wheel[deg]/1(Out1) -> Mux/3
  Angle_Beta_RR_Wheel[deg]/1(Out1) -> Mux/2
  Angle_Alpha_RR_Wheel[deg]/1(Out1) -> Mux/1
  Bus Selector2/14 -> Displ_Spring_RR[m]/1(In1)  "<Displ_Spring_Right[m]>"
  Bus Selector2/13 -> Angle_Gamma_RR_Wheel[deg]/1(In1)  "<Angle_Gamma_Right_Wheel[deg]>"
  Bus Selector2/12 -> Angle_Beta_RR_Wheel[deg]/1(In1)  "<Angle_Beta_Right_Wheel[deg]>"
  Bus Selector2/1 -> Pos_RL_Wheel[x;y;z][m]/1(In1)  "<Pos_Left_Wheel[x;y;z][m]>"
  Bus Selector/1 -> Pos_FL_Wheel[x;y;z][m]/1(In1)  "<Pos_Left_Wheel[x;y;z][m]>"
  Bus Selector1/4 -> Bus Selector4/1  "<SuspensionForcesRear>"
  Bus Selector1/3 -> Bus Selector2/1  "<SuspensionKinematicsRear>"
  Bus Selector1/2 -> Bus Selector3/1  "<SuspensionForcesFront>"
  Bus Selector1/1 -> Bus Selector/1  "<SuspensionKinematicsFront>"
  Bus Selector4/5 -> F_Stabilizer_Rear[N]/1(In1)  "<F_Stabilizer[N]>"
  Bus Selector4/4 -> F_RR_Damper[N]/1(In1)  "<F_RR_Damper[N]>"
  Bus Selector4/3 -> F_RR_Spring[N]/1(In1)  "<F_RR_Spring[N]>"
  Bus Selector4/2 -> F_RL_Damper[N]/1(In1)  "<F_RL_Damper[N]>"
  Bus Selector4/1 -> F_RL_Spring[N]/1(In1)  "<F_RL_Spring[N]>"
  Bus Selector2/16 -> Displ_Damper_RR_dt[m|s]/1(In1)  "<Displ_Damper_Right_dt[m|s]>"
  Bus Selector2/15 -> Displ_Damper_RR[m]/1(In1)  "<Displ_Damper_Right[m]>"
  Bus Selector2/11 -> Angle_Alpha_RR_Wheel[deg]/1(In1)  "<Angle_Alpha_Right_Wheel[deg]>"
  Bus Selector2/10 -> Angle_RR_Wheel[Alpha;Beta;Gamma][deg]/1(In1)  "<Angle_Right_Wheel[Alpha;Beta;Gamma][deg]>"
  Bus Selector2/8 -> Displ_Damper_RL_dt[m|s]/1(In1)  "<Displ_Damper_Left_dt[m|s]>"
  Bus Selector2/7 -> Displ_Damper_RL[m]/1(In1)  "<Displ_Damper_Left[m]>"
  Bus Selector2/6 -> Displ_Spring_RL[m]/1(In1)  "<Displ_Spring_Left[m]>"
  Bus Selector2/2 -> Angle_RL_Wheel[Alpha;Beta;Gamma][deg]/1(In1)  "<Angle_Left_Wheel[Alpha;Beta;Gamma][deg]>"
  Displ_Damper_RR_dt[m|s]/1(Out1) -> Kin_RR/5  "Displ_Damper_RR_dt[m|s]"
  Displ_Damper_RR[m]/1(Out1) -> Kin_RR/4  "Displ_Damper_RR[m]"
  Displ_Spring_RR[m]/1(Out1) -> Kin_RR/3  "Displ_Spring_RRm]"
  Pos_RR_Wheel[x;y;z][m]/1(Out1) -> Kin_RR/1  "Pos_RR_Wheel[x;y;z][m]"
  Displ_Stabilizer_Rear[m]/1(Out1) -> Kin_Stabi_Rear/1  "Displ_Stabilizer_Rear[m]"
  F_RL_Spring[N]/1(Out1) -> Force_Rear/1  "F_RL_Spring[N]"
  F_RL_Damper[N]/1(Out1) -> Force_Rear/2  "F_RL_Damper[N]"
  F_Stabilizer_Rear[N]/1(Out1) -> Force_Rear/5  "F_Stabilizer_Rear[N]"
  F_RR_Damper[N]/1(Out1) -> Force_Rear/4  "F_RR_Damper[N]"
  F_RR_Spring[N]/1(Out1) -> Force_Rear/3  "F_RR_Spring[N]"
  Displ_Damper_RL_dt[m|s]/1(Out1) -> Kin_RL/5  "Displ_Damper_RL_dt[m|s]"
  Displ_Damper_RL[m]/1(Out1) -> Kin_RL/4  "Displ_Damper_RL[m]"
  Displ_Spring_RL[m]/1(Out1) -> Kin_RL/3  "Displ_Spring_RL[m]"
  Pos_RL_Wheel[x;y;z][m]/1(Out1) -> Kin_RL/1  "Pos_RL_Wheel[x;y;z][m]"
  Displ_Damper_FR_dt[m|s]/1(Out1) -> Kin_FR/5  "Displ_Damper_FR_dt[m|s]"
  Displ_Damper_FR[m]/1(Out1) -> Kin_FR/4  "Displ_Damper_FR[m]"
  Displ_Spring_FRm]/1(Out1) -> Kin_FR/3  "Displ_Spring_FRm]"
  Pos_FR_Wheel[x;y;z][m]/1(Out1) -> Kin_FR/1  "Pos_FR_Wheel[x;y;z][m]"
  Displ_Stabilizer_Front[m]/1(Out1) -> Kin_Stabi_Front/1  "Displ_Stabilizer_Front[m]"
  F_FL_Spring[N]/1(Out1) -> Force_Front/1  "F_FL_Spring[N]"
  F_FL_Damper[N]/1(Out1) -> Force_Front/2  "F_FL_Damper[N]"
  F_Stabilizer_Front[N]/1(Out1) -> Force_Front/5  "F_Stabilizer_Front[N]"
  F_FR_Damper[N]/1(Out1) -> Force_Front/4  "F_FR_Damper[N]"
  F_FR_Spring[N]/1(Out1) -> Force_Front/3  "F_FR_Spring[N]"
  Bus Selector3/5 -> F_Stabilizer_Front[N]/1(In1)  "<F_Stabilizer[N]>"
  Bus Selector3/4 -> F_FR_Damper[N]/1(In1)  "<F_FR_Damper[N]>"
  Bus Selector3/3 -> F_FR_Spring[N]/1(In1)  "<F_FR_Spring[N]>"
  Bus Selector3/2 -> F_FL_Damper[N]/1(In1)  "<F_FL_Damper[N]>"
  Bus Selector3/1 -> F_FL_Spring[N]/1(In1)  "<F_FL_Spring[N]>"
  Displ_Damper_FL_dt[m|s]/1(Out1) -> Kin_FL/5  "Displ_Damper_FL_dt[m|s]"
  Displ_Damper_FL[m]/1(Out1) -> Kin_FL/4  "Displ_Damper_FL[m]"
  Displ_Spring_FL[m]/1(Out1) -> Kin_FL/3  "Displ_Spring_FL[m]"
  Pos_FL_Wheel[x;y;z][m]/1(Out1) -> Kin_FL/1  "Pos_FL_Wheel[x;y;z][m]"
  Suspension/1 -> Bus Selector1/1
  Bus Selector2/17 -> Displ_Stabilizer_Rear[m]/1(In1)  "<Displ_Stabilizer[m]>"
  Bus Selector2/9 -> Pos_RR_Wheel[x;y;z][m]/1(In1)  "<Pos_Right_Wheel[x;y;z][m]>"

== system ASM_Traffic_new/VehicleDynamics/Plant/UserInterface/DISP_Plant/Tire ==
  Tire : Inport
  Bus Selector2 : BusSelector  OutputSignals=Tire_allSignals.Tire_FL.Tire.Slip_x[],Tire_allSignals.Tire_FR.Tire.Slip_x[],Tire_allSignals.Tire_RL.Tire.Slip_x[],Tire_allSignals.Tire_RR.Tire.Slip_x[],Tire_allSignals.Tire_FL.Tire.Slip_y[],Tire_allSignals.Tire_FR.Tire.Slip_y[],Tire_allSignals.Tire_RL.Tire.Slip_y[],Tire_allSignals.Tire_RR.Tire.Slip_y[],Tire_allSignals.Tire_FL.Tire.r_Dyn_Tire[m],Tire_allSignals.Tire_FR.Tire.r_Dyn_Tire[m],Tire_allSignals.Tire_RL.Tire.r_Dyn_Tire[m],Tire_allSignals.Tire_RR.Tire.r_Dyn_Tire[m],Tire_allSignals.Tire_FL.Tire.F_x_Dyn_Tire_CoorSys_CP[N],Tire_allSignals.Tire_FR.Tire.F_x_Dyn_Tire_CoorSys_CP[N],Tire_allSignals.Tire_RL.Tire.F_x_Dyn_Tire_CoorSys_CP[N],Tire_allSignals.Tire_RR.Tire.F_x_Dyn_Tire_CoorSys_CP[N],Tire_allSignals.Tire_FL.Tire.F_y_Dyn_Tire_CoorSys_CP[N],Tire_allSignals.Tire_FR.Tire.F_y_Dyn_Tire_CoorSys_CP[N],Tire_allSignals.Tire_RL.Tire.F_y_Dyn_Tire_CoorSys_CP[N],Tire_allSignals.Tire_RR.Tire.F_y_Dyn_Tire_CoorSys_CP[N],Tire_allSignals.Tire_FL.Tire.F_z_Dyn_Tire_CoorSys_CP[N],Tire_allSignals.Tire_FR.Tire.F_z_Dyn_Tire_CoorSys_CP[N],Tire_allSignals.Tire_RL.Tire.F_z_Dyn_Tire_CoorSys_CP[N],Tire_allSignals.Tire_RR.Tire.F_z_Dyn_Tire_CoorSys_CP[N],Tire_allSignals.Tire_FL.Tire.Trq_x_CoorSys_CP[Nm],Tire_allSignals.Tire_FR.Tire.Trq_x_CoorSys_CP[Nm],Tire_allSignals.Tire_RL.Tire.Trq_x_CoorSys_CP[Nm],Tire_allSignals.Tire_RR.Tire.Trq_x_CoorSys_CP[Nm],Tire_allSignals.Tire_FL.Tire.Trq_y_CoorSys_W[Nm],Tire_allSignals.Tire_FR.Tire.Trq_y_CoorSys_W[Nm],Tire_allSignals.Tire_RL.Tire.Trq_y_CoorSys_W[Nm],Tire_allSignals.Tire_RR.Tire.Trq_y_CoorSys_W[Nm],Tire_allSignals.Tire_FL.Tire.Trq_z_CoorSys_CP[Nm],Tire_allSignals.Tire_FR.Tire.Trq_z_CoorSys_CP[Nm],Tire_allSignals.Tire_RL.Tire.Trq_z_CoorSys_CP[Nm],Tire_allSignals.Tire_RR.Tire.Trq_z_CoorSys_CP[Nm],Tire_allSignals.Tire_FL.Tire.v_Circumf_Dyn_Wheel[km|h],Tire_allSignals.Tire_FR.Tire.v_Circumf_Dyn_Wheel[km|h],Tire_allSignals.Tire_RL.Tire.v_Circumf_Dyn_Wheel[km|h],Tire_allSignals.Tire_RR.Tire.v_Circumf_Dyn_Wheel[km|h]
  DynamicRadius : Scope  NumInputPorts=4
  F_x_Dyn_FL_Tire_CoorSys_CP[N] : Subsystem
      mask Display: disp('')
  F_x_Dyn_FR_Tire_CoorSys_CP[N] : Subsystem
      mask Display: disp('')
  F_x_Dyn_RL_Tire_CoorSys_CP[N] : Subsystem
      mask Display: disp('')
  F_x_Dyn_RR_Tire_CoorSys_CP[N] : Subsystem
      mask Display: disp('')
  F_y_Dyn_FL_Tire_CoorSys_CP[N] : Subsystem
      mask Display: disp('')
  F_y_Dyn_FR_Tire_CoorSys_CP[N] : Subsystem
      mask Display: disp('')
  F_y_Dyn_RL_Tire_CoorSys_CP[N] : Subsystem
      mask Display: disp('')
  F_y_Dyn_RR_Tire_CoorSys_CP[N] : Subsystem
      mask Display: disp('')
  F_z_Dyn_FL_Tire_CoorSys_CP[N] : Subsystem
      mask Display: disp('')
  F_z_Dyn_FR_Tire_CoorSys_CP[N] : Subsystem
      mask Display: disp('')
  F_z_Dyn_RL_Tire_CoorSys_CP[N] : Subsystem
      mask Display: disp('')
  F_z_Dyn_RR_Tire_CoorSys_CP[N] : Subsystem
      mask Display: disp('')
  Mux{,1..7} (8 alike) : Mux
  Slip : Scope  NumInputPorts=2
  Slip_x_FL[] : Subsystem
      mask Display: disp('')
  Slip_x_FR[] : Subsystem
      mask Display: disp('')
  Slip_x_RL[] : Subsystem
      mask Display: disp('')
  Slip_x_RR[] : Subsystem
      mask Display: disp('')
  Slip_y_FL[] : Subsystem
      mask Display: disp('')
  Slip_y_FR[] : Subsystem
      mask Display: disp('')
  Slip_y_RL[] : Subsystem
      mask Display: disp('')
  Slip_y_RR[] : Subsystem
      mask Display: disp('')
  TireCircumfSpeed : Scope  NumInputPorts=4
  TireForce : Scope  NumInputPorts=3
  TireTorque : Scope  NumInputPorts=3
  Trq_x_FL_CoorSys_CP[Nm] : Subsystem
      mask Display: disp('')
  Trq_x_FR_CoorSys_CP[Nm] : Subsystem
      mask Display: disp('')
  Trq_x_RL_CoorSys_CP[Nm] : Subsystem
      mask Display: disp('')
  Trq_x_RR_CoorSys_CP[Nm] : Subsystem
      mask Display: disp('')
  Trq_y_FL_CoorSys_W[Nm] : Subsystem
      mask Display: disp('')
  Trq_y_FR_CoorSys_W[Nm] : Subsystem
      mask Display: disp('')
  Trq_y_RL_CoorSys_W[Nm] : Subsystem
      mask Display: disp('')
  Trq_y_RR_CoorSys_W[Nm] : Subsystem
      mask Display: disp('')
  Trq_z_FL_CoorSys_CP[Nm] : Subsystem
      mask Display: disp('')
  Trq_z_FR_CoorSys_CP[Nm] : Subsystem
      mask Display: disp('')
  Trq_z_RL_CoorSys_CP[Nm] : Subsystem
      mask Display: disp('')
  Trq_z_RR_CoorSys_CP[Nm] : Subsystem
      mask Display: disp('')
  r_Dyn_FL_Tire[m] : Subsystem
      mask Display: disp('')
  r_Dyn_FR_Tire[m] : Subsystem
      mask Display: disp('')
  r_Dyn_RL_Tire[m] : Subsystem
      mask Display: disp('')
  r_Dyn_RR_Tire[m] : Subsystem
      mask Display: disp('')
  v_Circumf_Dyn_FL_Wheel[km|h] : Subsystem
      mask Display: disp('')
  v_Circumf_Dyn_FR_Wheel[km|h] : Subsystem
      mask Display: disp('')
  v_Circumf_Dyn_RL_Wheel[km|h] : Subsystem
      mask Display: disp('')
  v_Circumf_Dyn_RR_Wheel[km|h] : Subsystem
      mask Display: disp('')
  wires:
  Mux7/1 -> Slip/2  "Slip_y[]"
  Mux6/1 -> Slip/1  "Slip_x[]"
  Mux5/1 -> TireTorque/3  "Trq_z[Nm]"
  Mux3/1 -> TireTorque/2  "Trq_y[Nm]"
  Mux4/1 -> TireTorque/1  "Trq_x[Nm]"
  Mux2/1 -> TireForce/3  "F_z[N]"
  Mux/1 -> TireForce/2  "F_y[N]"
  Mux1/1 -> TireForce/1  "F_x[N]"
  Tire/1 -> Bus Selector2/1
  Slip_x_FL[]/1(Out1) -> Mux6/1  "Slip_x_FL[]"
  Slip_x_FR[]/1(Out1) -> Mux6/2  "Slip_x_FR[]"
  Slip_x_RL[]/1(Out1) -> Mux6/3  "Slip_x_RL[]"
  Slip_x_RR[]/1(Out1) -> Mux6/4  "Slip_x_RR[]"
  Slip_y_FL[]/1(Out1) -> Mux7/1  "Slip_y_FL[]"
  Slip_y_FR[]/1(Out1) -> Mux7/2  "Slip_y_FR[]"
  Slip_y_RL[]/1(Out1) -> Mux7/3  "Slip_y_RL[]"
  Slip_y_RR[]/1(Out1) -> Mux7/4  "Slip_y_RR[]"
  Bus Selector2/1 -> Slip_x_FL[]/1(In1)  "<Slip_x[]>"
  Bus Selector2/2 -> Slip_x_FR[]/1(In1)  "<Slip_x[]>"
  Bus Selector2/3 -> Slip_x_RL[]/1(In1)  "<Slip_x[]>"
  Bus Selector2/4 -> Slip_x_RR[]/1(In1)  "<Slip_x[]>"
  Bus Selector2/5 -> Slip_y_FL[]/1(In1)  "<Slip_y[]>"
  Bus Selector2/6 -> Slip_y_FR[]/1(In1)  "<Slip_y[]>"
  Bus Selector2/7 -> Slip_y_RL[]/1(In1)  "<Slip_y[]>"
  Bus Selector2/8 -> Slip_y_RR[]/1(In1)  "<Slip_y[]>"
  Trq_x_FL_CoorSys_CP[Nm]/1(Out1) -> Mux4/1  "Trq_x_FL_CoorSys_CP[Nm]"
  Trq_x_FR_CoorSys_CP[Nm]/1(Out1) -> Mux4/2  "Trq_x_FR_CoorSys_CP[Nm]"
  Trq_x_RL_CoorSys_CP[Nm]/1(Out1) -> Mux4/3  "Trq_x_RL_CoorSys_CP[Nm]"
  Trq_x_RR_CoorSys_CP[Nm]/1(Out1) -> Mux4/4  "Trq_x_RR_CoorSys_CP[Nm]"
  Trq_y_FL_CoorSys_W[Nm]/1(Out1) -> Mux3/1  "Trq_y_FL_CoorSys_W[Nm]"
  Trq_y_FR_CoorSys_W[Nm]/1(Out1) -> Mux3/2  "Trq_y_FR_CoorSys_W[Nm]"
  Trq_y_RL_CoorSys_W[Nm]/1(Out1) -> Mux3/3  "Trq_y_RL_CoorSys_W[Nm]"
  Trq_y_RR_CoorSys_W[Nm]/1(Out1) -> Mux3/4  "Trq_y_RR_CoorSys_W[Nm]"
  Trq_z_FL_CoorSys_CP[Nm]/1(Out1) -> Mux5/1  "Trq_z_FL_CoorSys_CP[Nm]"
  Trq_z_FR_CoorSys_CP[Nm]/1(Out1) -> Mux5/2  "Trq_z_FR_CoorSys_CP[Nm]"
  Trq_z_RL_CoorSys_CP[Nm]/1(Out1) -> Mux5/3  "Trq_z_RL_CoorSys_CP[Nm]"
  Trq_z_RR_CoorSys_CP[Nm]/1(Out1) -> Mux5/4  "Trq_z_RR_CoorSys_CP[Nm]"
  F_x_Dyn_FL_Tire_CoorSys_CP[N]/1(Out1) -> Mux1/1  "F_x_Dyn_FL_Tire_CoorSys_CP[N]"
  F_x_Dyn_FR_Tire_CoorSys_CP[N]/1(Out1) -> Mux1/2  "F_x_Dyn_FR_Tire_CoorSys_CP[N]"
  F_x_Dyn_RL_Tire_CoorSys_CP[N]/1(Out1) -> Mux1/3  "F_x_Dyn_RL_Tire_CoorSys_CP[N]"
  F_x_Dyn_RR_Tire_CoorSys_CP[N]/1(Out1) -> Mux1/4  "F_x_Dyn_RR_Tire_CoorSys_CP[N]"
  F_y_Dyn_FL_Tire_CoorSys_CP[N]/1(Out1) -> Mux/1  "F_y_Dyn_FL_Tire_CoorSys_CP[N]"
  F_y_Dyn_FR_Tire_CoorSys_CP[N]/1(Out1) -> Mux/2  "F_y_Dyn_FR_Tire_CoorSys_CP[N]"
  F_y_Dyn_RL_Tire_CoorSys_CP[N]/1(Out1) -> Mux/3  "F_y_Dyn_RL_Tire_CoorSys_CP[N]"
  F_y_Dyn_RR_Tire_CoorSys_CP[N]/1(Out1) -> Mux/4  "F_y_Dyn_RR_Tire_CoorSys_CP[N]"
  F_z_Dyn_FL_Tire_CoorSys_CP[N]/1(Out1) -> Mux2/1  "F_z_Dyn_FL_Tire_CoorSys_CP[N]"
  F_z_Dyn_FR_Tire_CoorSys_CP[N]/1(Out1) -> Mux2/2  "F_z_Dyn_FR_Tire_CoorSys_CP[N]"
  F_z_Dyn_RL_Tire_CoorSys_CP[N]/1(Out1) -> Mux2/3  "F_z_Dyn_RL_Tire_CoorSys_CP[N]"
  F_z_Dyn_RR_Tire_CoorSys_CP[N]/1(Out1) -> Mux2/4  "F_z_Dyn_RR_Tire_CoorSys_CP[N]"
  v_Circumf_Dyn_FL_Wheel[km|h]/1(Out1) -> TireCircumfSpeed/1  "v_Circumf_Dyn_FL_Wheel[km|h]"
  v_Circumf_Dyn_FR_Wheel[km|h]/1(Out1) -> TireCircumfSpeed/2  "v_Circumf_Dyn_FR_Wheel[km|h]"
  v_Circumf_Dyn_RL_Wheel[km|h]/1(Out1) -> TireCircumfSpeed/3  "v_Circumf_Dyn_RL_Wheel[km|h]"
  v_Circumf_Dyn_RR_Wheel[km|h]/1(Out1) -> TireCircumfSpeed/4  "v_Circumf_Dyn_RR_Wheel[km|h]"
  r_Dyn_FL_Tire[m]/1(Out1) -> DynamicRadius/1  "r_Dyn_FL_Tire[m]"
  r_Dyn_FR_Tire[m]/1(Out1) -> DynamicRadius/2  "r_Dyn_FR_Tire[m]"
  r_Dyn_RL_Tire[m]/1(Out1) -> DynamicRadius/3  "r_Dyn_RL_Tire[m]"
  r_Dyn_RR_Tire[m]/1(Out1) -> DynamicRadius/4  "r_Dyn_RR_Tire[m]"
  Bus Selector2/9 -> r_Dyn_FL_Tire[m]/1(In1)  "<r_Dyn_Tire[m]>"
  Bus Selector2/10 -> r_Dyn_FR_Tire[m]/1(In1)  "<r_Dyn_Tire[m]>"
  Bus Selector2/11 -> r_Dyn_RL_Tire[m]/1(In1)  "<r_Dyn_Tire[m]>"
  Bus Selector2/12 -> r_Dyn_RR_Tire[m]/1(In1)  "<r_Dyn_Tire[m]>"
  Bus Selector2/13 -> F_x_Dyn_FL_Tire_CoorSys_CP[N]/1(In1)  "<F_x_Dyn_Tire_CoorSys_CP[N]>"
  Bus Selector2/14 -> F_x_Dyn_FR_Tire_CoorSys_CP[N]/1(In1)  "<F_x_Dyn_Tire_CoorSys_CP[N]>"
  Bus Selector2/15 -> F_x_Dyn_RL_Tire_CoorSys_CP[N]/1(In1)  "<F_x_Dyn_Tire_CoorSys_CP[N]>"
  Bus Selector2/16 -> F_x_Dyn_RR_Tire_CoorSys_CP[N]/1(In1)  "<F_x_Dyn_Tire_CoorSys_CP[N]>"
  Bus Selector2/17 -> F_y_Dyn_FL_Tire_CoorSys_CP[N]/1(In1)  "<F_y_Dyn_Tire_CoorSys_CP[N]>"
  Bus Selector2/18 -> F_y_Dyn_FR_Tire_CoorSys_CP[N]/1(In1)  "<F_y_Dyn_Tire_CoorSys_CP[N]>"
  Bus Selector2/19 -> F_y_Dyn_RL_Tire_CoorSys_CP[N]/1(In1)  "<F_y_Dyn_Tire_CoorSys_CP[N]>"
  Bus Selector2/20 -> F_y_Dyn_RR_Tire_CoorSys_CP[N]/1(In1)  "<F_y_Dyn_Tire_CoorSys_CP[N]>"
  Bus Selector2/21 -> F_z_Dyn_FL_Tire_CoorSys_CP[N]/1(In1)  "<F_z_Dyn_Tire_CoorSys_CP[N]>"
  Bus Selector2/22 -> F_z_Dyn_FR_Tire_CoorSys_CP[N]/1(In1)  "<F_z_Dyn_Tire_CoorSys_CP[N]>"
  Bus Selector2/23 -> F_z_Dyn_RL_Tire_CoorSys_CP[N]/1(In1)  "<F_z_Dyn_Tire_CoorSys_CP[N]>"
  Bus Selector2/24 -> F_z_Dyn_RR_Tire_CoorSys_CP[N]/1(In1)  "<F_z_Dyn_Tire_CoorSys_CP[N]>"
  Bus Selector2/25 -> Trq_x_FL_CoorSys_CP[Nm]/1(In1)  "<Trq_x_CoorSys_CP[Nm]>"
  Bus Selector2/26 -> Trq_x_FR_CoorSys_CP[Nm]/1(In1)  "<Trq_x_CoorSys_CP[Nm]>"
  Bus Selector2/27 -> Trq_x_RL_CoorSys_CP[Nm]/1(In1)  "<Trq_x_CoorSys_CP[Nm]>"
  Bus Selector2/28 -> Trq_x_RR_CoorSys_CP[Nm]/1(In1)  "<Trq_x_CoorSys_CP[Nm]>"
  Bus Selector2/29 -> Trq_y_FL_CoorSys_W[Nm]/1(In1)  "<Trq_y_CoorSys_W[Nm]>"
  Bus Selector2/30 -> Trq_y_FR_CoorSys_W[Nm]/1(In1)  "<Trq_y_CoorSys_W[Nm]>"
  Bus Selector2/31 -> Trq_y_RL_CoorSys_W[Nm]/1(In1)  "<Trq_y_CoorSys_W[Nm]>"
  Bus Selector2/32 -> Trq_y_RR_CoorSys_W[Nm]/1(In1)  "<Trq_y_CoorSys_W[Nm]>"
  Bus Selector2/33 -> Trq_z_FL_CoorSys_CP[Nm]/1(In1)  "<Trq_z_CoorSys_CP[Nm]>"
  Bus Selector2/34 -> Trq_z_FR_CoorSys_CP[Nm]/1(In1)  "<Trq_z_CoorSys_CP[Nm]>"
  Bus Selector2/35 -> Trq_z_RL_CoorSys_CP[Nm]/1(In1)  "<Trq_z_CoorSys_CP[Nm]>"
  Bus Selector2/36 -> Trq_z_RR_CoorSys_CP[Nm]/1(In1)  "<Trq_z_CoorSys_CP[Nm]>"
  Bus Selector2/37 -> v_Circumf_Dyn_FL_Wheel[km|h]/1(In1)  "<v_Circumf_Dyn_Wheel[km|h]>"
  Bus Selector2/38 -> v_Circumf_Dyn_FR_Wheel[km|h]/1(In1)  "<v_Circumf_Dyn_Wheel[km|h]>"
  Bus Selector2/39 -> v_Circumf_Dyn_RL_Wheel[km|h]/1(In1)  "<v_Circumf_Dyn_Wheel[km|h]>"
  Bus Selector2/40 -> v_Circumf_Dyn_RR_Wheel[km|h]/1(In1)  "<v_Circumf_Dyn_Wheel[km|h]>"

== system ASM_Traffic_new/VehicleDynamics/Plant/UserInterface/DISP_Plant/Velocities ==
  Velocities : Inport
  Angle_SideSlip_Vehicle[deg] : Subsystem
      mask Display: disp('')
  AngularVelocities : Scope  NumInputPorts=3
  Bus Selector2 : BusSelector  OutputSignals=Vehicle.Linear.v_Vehicle_CoG[x;y;z][km|h].v_x_Vehicle_CoG[km|h],Vehicle.Linear.v_Vehicle_CoG[x;y;z][km|h].v_y_Vehicle_CoG[km|h],Vehicle.Linear.v_Vehicle_CoG[x;y;z][km|h].v_z_Vehicle_CoG[km|h],Vehicle.Linear.Angle_SideSlip_Vehicle[deg],Vehicle.Angular.w_Vehicle_CoG[x;y;z][deg|s].RollRate_Vehicle_CoG[deg|s],Vehicle.Angular.w_Vehicle_CoG[x;y;z][deg|s].PitchRate_Vehicle_CoG[deg|s],Vehicle.Angular.w_Vehicle_CoG[x;y;z][deg|s].YawRate_Vehicle_CoG[deg|s]
  PitchRate_Vehicle_CoG[deg|s] : Subsystem
      mask Display: disp('')
  RollRate_Vehicle_CoG[deg|s] : Subsystem
      mask Display: disp('')
  TransVelocities : Scope  NumInputPorts=4
  YawRate_Vehicle_CoG[deg|s] : Subsystem
      mask Display: disp('')
  v_x_Vehicle_CoG[km|h] : Subsystem
      mask Display: disp('')
  v_y_Vehicle_CoG[km|h] : Subsystem
      mask Display: disp('')
  v_z_Vehicle_CoG[km|h] : Subsystem
      mask Display: disp('')
  wires:
  Velocities/1 -> Bus Selector2/1
  RollRate_Vehicle_CoG[deg|s]/1(Out1) -> AngularVelocities/1  "RollRate_Vehicle_CoG[deg|s]"
  PitchRate_Vehicle_CoG[deg|s]/1(Out1) -> AngularVelocities/2  "PitchRate_Vehicle_CoG[deg|s]"
  YawRate_Vehicle_CoG[deg|s]/1(Out1) -> AngularVelocities/3  "YawRate_Vehicle_CoG[deg|s]"
  v_x_Vehicle_CoG[km|h]/1(Out1) -> TransVelocities/1  "v_x_Vehicle_CoG[km|h]"
  v_y_Vehicle_CoG[km|h]/1(Out1) -> TransVelocities/2  "v_y_Vehicle_CoG[km|h]"
  v_z_Vehicle_CoG[km|h]/1(Out1) -> TransVelocities/3  "v_z_Vehicle_CoG[km|h]"
  Angle_SideSlip_Vehicle[deg]/1(Out1) -> TransVelocities/4  "Angle_SideSlip_Vehicle[deg]"
  Bus Selector2/1 -> v_x_Vehicle_CoG[km|h]/1(In1)  "<v_x_Vehicle_CoG[km|h]>"
  Bus Selector2/2 -> v_y_Vehicle_CoG[km|h]/1(In1)  "<v_y_Vehicle_CoG[km|h]>"
  Bus Selector2/3 -> v_z_Vehicle_CoG[km|h]/1(In1)  "<v_z_Vehicle_CoG[km|h]>"
  Bus Selector2/4 -> Angle_SideSlip_Vehicle[deg]/1(In1)  "<Angle_SideSlip_Vehicle[deg]>"
  Bus Selector2/5 -> RollRate_Vehicle_CoG[deg|s]/1(In1)  "<RollRate_Vehicle_CoG[deg|s]>"
  Bus Selector2/6 -> PitchRate_Vehicle_CoG[deg|s]/1(In1)  "<PitchRate_Vehicle_CoG[deg|s]>"
  Bus Selector2/7 -> YawRate_Vehicle_CoG[deg|s]/1(In1)  "<YawRate_Vehicle_CoG[deg|s]>"

== system ASM_Traffic_new/VehicleDynamics/Plant/UserInterface/DISP_Plant/WheelSpeeds ==
  WheelSpeeds : Inport
  Bus Selector2 : BusSelector  OutputSignals=WheelSpeed.omega_FL_Wheel[rad|s],WheelSpeed.omega_FR_Wheel[rad|s],WheelSpeed.omega_RL_Wheel[rad|s],WheelSpeed.omega_RR_Wheel[rad|s]
  WheelSpeeds1 : Scope  NumInputPorts=4
  omega_FL_Wheel[rad|s] : Subsystem
      mask Display: disp('')
  omega_FR_Wheel[rad|s] : Subsystem
      mask Display: disp('')
  omega_RL_Wheel[rad|s] : Subsystem
      mask Display: disp('')
  omega_RR_Wheel[rad|s] : Subsystem
      mask Display: disp('')
  wires:
  omega_RR_Wheel[rad|s]/1(Out1) -> WheelSpeeds1/4  "omega_RR_Wheel[rad|s]"
  omega_RL_Wheel[rad|s]/1(Out1) -> WheelSpeeds1/3  "omega_RL_Wheel[rad|s]"
  omega_FR_Wheel[rad|s]/1(Out1) -> WheelSpeeds1/2  "omega_FR_Wheel[rad|s]"
  omega_FL_Wheel[rad|s]/1(Out1) -> WheelSpeeds1/1  "omega_FL_Wheel[rad|s]"
  WheelSpeeds/1 -> Bus Selector2/1
  Bus Selector2/1 -> omega_FL_Wheel[rad|s]/1(In1)  "<omega_FL_Wheel[rad|s]>"
  Bus Selector2/2 -> omega_FR_Wheel[rad|s]/1(In1)  "<omega_FR_Wheel[rad|s]>"
  Bus Selector2/3 -> omega_RL_Wheel[rad|s]/1(In1)  "<omega_RL_Wheel[rad|s]>"
  Bus Selector2/4 -> omega_RR_Wheel[rad|s]/1(In1)  "<omega_RR_Wheel[rad|s]>"

== system ASM_Traffic_new/VehicleDynamics/Plant/UserInterface/PAR_Plant/BrakeHydraulics_DistributionPattern_Switch ==
  Sw_DistributionPattern[1X|2II] : Constant
  Sw_DistributionPattern_[1X|2II] : Outport  VectorParamsAs1DForOutWhenUnconnected=off
  wires:
  Sw_DistributionPattern[1X|2II]/1 -> Sw_DistributionPattern_[1X|2II]/1  "Sw_DistributionPattern_[1X|2II]"

== system ASM_Traffic_new/VehicleDynamics/Plant/UserInterface/PAR_Plant/Suspension_Inits ==
  Bus Creator1 : BusCreator  Inputs=2
  Mux : Mux
  Mux2 : Mux
  z_FL_Init[m] : Constant  Value=0  VectorParams1D=off
  z_FL_Init_dt[m|s] : Constant  Value=0  VectorParams1D=off
  z_FR_Init[m] : Constant  Value=0  VectorParams1D=off
  z_FR_Init_dt[m|s] : Constant  Value=0  VectorParams1D=off
  z_RL_Init[m] : Constant  Value=0  VectorParams1D=off
  z_RL_Init_dt[m|s] : Constant  Value=0  VectorParams1D=off
  z_RR_Init[m] : Constant  Value=0  VectorParams1D=off
  z_RR_Init_dt[m|s] : Constant  Value=0  VectorParams1D=off
  Suspension_Init : Outport  VectorParamsAs1DForOutWhenUnconnected=off
  wires:
  Mux2/1 -> Bus Creator1/1  "q_dt_Wheel_Init[:]"
  Mux/1 -> Bus Creator1/2  "q_Wheel_Init[:]"
  Bus Creator1/1 -> Suspension_Init/1  "Suspension_Init"
  z_FL_Init_dt[m|s]/1 -> Mux2/1
  z_FR_Init_dt[m|s]/1 -> Mux2/2
  z_RL_Init_dt[m|s]/1 -> Mux2/3
  z_RR_Init_dt[m|s]/1 -> Mux2/4
  z_FL_Init[m]/1 -> Mux/1
  z_FR_Init[m]/1 -> Mux/2
  z_RL_Init[m]/1 -> Mux/3
  z_RR_Init[m]/1 -> Mux/4

== system ASM_Traffic_new/VehicleDynamics/Plant/UserInterface/PAR_Plant/Tire_Switches ==
  Bus Creator1 : BusCreator  Inputs=2
  Sw_r_Tire[1:intern;2:extern] : Constant  VectorParams1D=off
  r_Tire_extern[m] : Constant  Value=0.31  VectorParams1D=off
  Tire_Switches : Outport  VectorParamsAs1DForOutWhenUnconnected=off
  wires:
  Bus Creator1/1 -> Tire_Switches/1
  Sw_r_Tire[1:intern;2:extern]/1 -> Bus Creator1/1  "Sw_r_Tire[1:intern;2:extern]"
  r_Tire_extern[m]/1 -> Bus Creator1/2  "r_Tire_extern[m]"

== system ASM_Traffic_new/VehicleDynamics/Plant/VehicleDynamics/ASMSignalCollector/Driving_Resistances ==
  F_Vehicle_Gravitational[x;y;z][N] : Inport
  Coef_RollingRes_Mean[] : Inport  Port=2
  F_x_Aero_CoorSys_V[N] : Inport  Port=3
  Bus Creator : BusCreator  Inputs=1
  Gain : Gain  Gain=-1
  Gain1 : Gain
  Gain2 : Gain
  Product : Product
  Sum : Sum  Inputs=+++
  X_Component : Selector  InputPortWidth=3  IndexOptions=Index vector (dialog)  Indices=[1]  OutputSizes=1
  Z_Component : Selector  InputPortWidth=3  IndexOptions=Index vector (dialog)  Indices=[3]  OutputSizes=1
  F_Driving_Res[N] : Outport  VectorParamsAs1DForOutWhenUnconnected=off
  wires:
  Gain/1 -> Bus Creator/1  "F_Driving_Res[N]"
  Sum/1 -> Gain/1
  Gain1/1 -> Sum/2  "F_Slope[N]"
  Gain2/1 -> Sum/1  "F_Aerodynamics[N]"
  Product/1 -> Sum/3  "F_Roll[N]"
  X_Component/1 -> Gain1/1
  Z_Component/1 -> Product/1
  Coef_RollingRes_Mean[]/1 -> Product/2
  F_x_Aero_CoorSys_V[N]/1 -> Gain2/1
  F_Vehicle_Gravitational[x;y;z][N]/1 -> Z_Component/1, X_Component/1
  Bus Creator/1 -> F_Driving_Res[N]/1  "DrivingResistances"

== system ASM_Traffic_new/VehicleDynamics/Plant/VehicleDynamics/Brake/ASMSignalCollector ==
  BusCreator3 : BusCreator  Inputs=5
  ASMSignalBus : Outport  VectorParamsAs1DForOutWhenUnconnected=off
  wires:
  [ASMBUS_VehicleDynamics_Manifold] -> BusCreator3/5
  [ASMBUS_VehicleDynamics_VacuumServo] -> BusCreator3/4
  [ASMBUS_VehicleDynamics_BrakeDisc] -> BusCreator3/3
  [TAG_DISP_BrkHyd_MasterBrakeCylinder] -> BusCreator3/1
  [ASMBUS_VehicleDynamics_BrakeHydraulics] -> BusCreator3/2
  BusCreator3/1 -> ASMSignalBus/1  "Brake"
